simulink model "pfc_analog_test"  (R2021b)
settings: Solver=ode45  StartTime=0.0  StopTime=p.duration  MaxStep=p.max_step  RelTol=1e-8  AbsTol=1e-10
values from neighbouring files (symbols this model uses):
  config = [10 1514 1000]    [validate_m1.m]
  event_file = fullfile(folder,[name '_events.csv'])    [event_case.m]    (also in pfc_case.m)
  p = pfc_parameters();p.duration=0.08;p.load_step_time=1    [probe_closed_loop.m]    (also in validate_analog.m = pfc_parameters();p.duration=40e-6;p.max_step=2e-6; validate_control_reset.m = pfc_parameters())
settings Model: Creator=yangs  LastModifiedBy=yangs
settings SolverCC: ZeroCrossControl=EnableAll  ZeroCrossAlgorithm=Adaptive

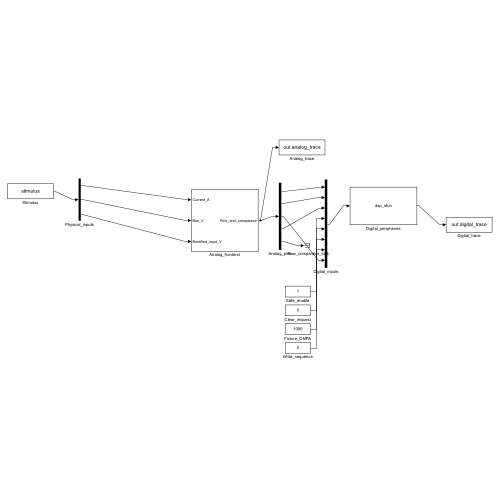
[thumbnail: Simulink's stored preview of the top-level diagram]
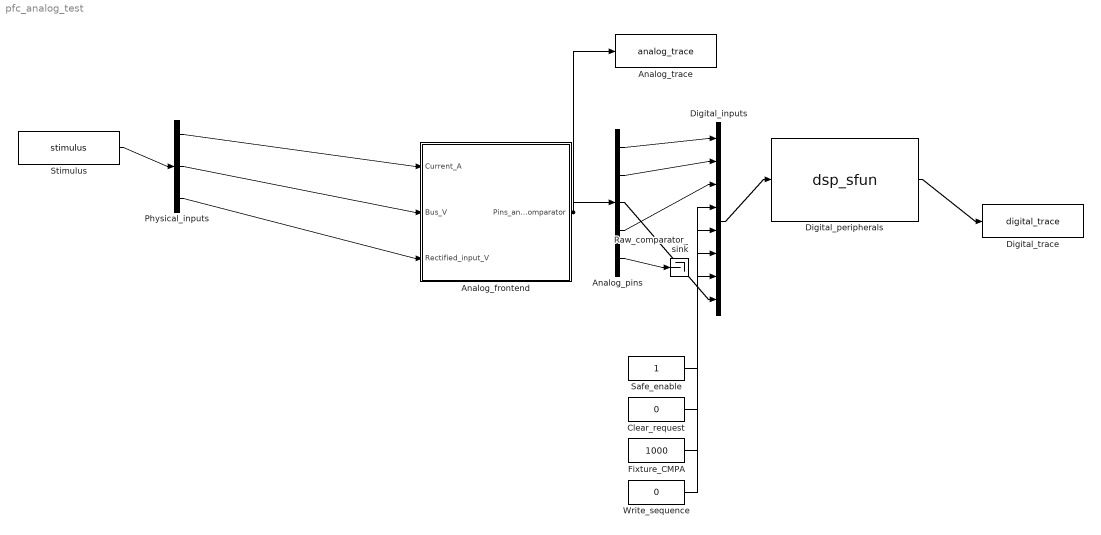
== system pfc_analog_test ==
  Analog_frontend : Subsystem
  Analog_pins : Demux  Outputs=5
  Analog_trace : ToWorkspace  VariableName=analog_trace  SaveFormat=Structure With Time  SampleTime=-1
  Clear_request : Constant  Value=0
  Digital_inputs : Mux  Inputs=8
  Digital_peripherals : S-Function  FunctionName=dsp_sfun  Parameters=config,event_file  SFunctionDeploymentMode=off  EnableBusSupport=off
  Digital_trace : ToWorkspace  VariableName=digital_trace  SaveFormat=Structure With Time  SampleTime=-1
  Fixture_CMPA : Constant  Value=1000
  Physical_inputs : Demux  Outputs=3
  Raw_comparator_sink : Terminator
  Safe_enable : Constant
  Stimulus : FromWorkspace  VariableName=stimulus  Interpolate=off  OutputAfterFinalValue=Holding final value
  Write_sequence : Constant  Value=0
  wires:
  Stimulus/1 -> Physical_inputs/1
  Analog_frontend/1(Pins_and_comparator) -> Analog_pins/1, Analog_trace/1
  Analog_pins/1 -> Digital_inputs/1
  Analog_pins/2 -> Digital_inputs/2
  Analog_pins/4 -> Digital_inputs/3
  Analog_pins/3 -> Digital_inputs/8
  Safe_enable/1 -> Digital_inputs/4
  Clear_request/1 -> Digital_inputs/5
  Fixture_CMPA/1 -> Digital_inputs/6
  Write_sequence/1 -> Digital_inputs/7
  Analog_pins/5 -> Raw_comparator_sink/1
  Digital_inputs/1 -> Digital_peripherals/1
  Digital_peripherals/1 -> Digital_trace/1
  Physical_inputs/1 -> Analog_frontend/1(Current_A)
  Physical_inputs/2 -> Analog_frontend/2(Bus_V)
  Physical_inputs/3 -> Analog_frontend/3(Rectified_input_V)

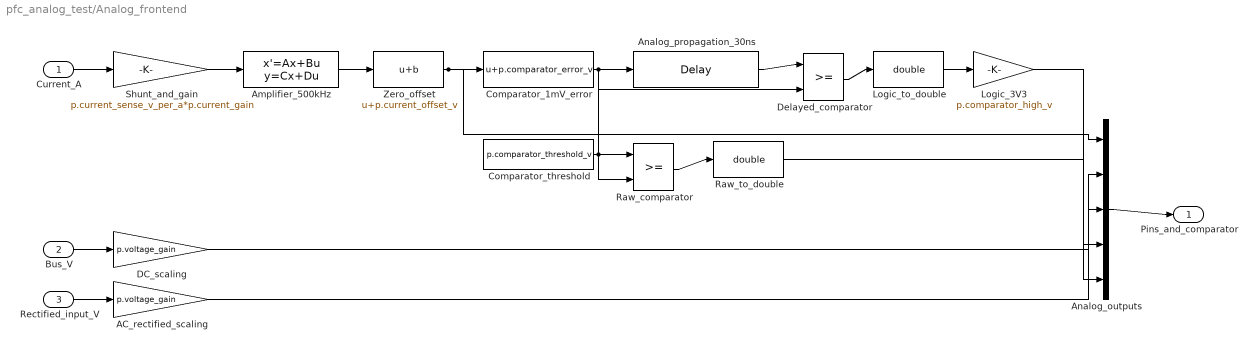
== system pfc_analog_test/Analog_frontend ==
  Current_A : Inport
  Bus_V : Inport  Port=2
  Rectified_input_V : Inport  Port=3
  AC_rectified_scaling : Gain  Gain=p.voltage_gain
  Amplifier_500kHz : StateSpace  A=-1/p.current_tau  B=1/p.current_tau  D=0  InitialCondition=0
  Analog_outputs : Mux  Inputs=5
  Analog_propagation_30ns : TransportDelay  DelayTime=p.comparator_delay_s
  Comparator_1mV_error : Bias  Bias=p.comparator_error_v
  Comparator_threshold : Constant  Value=p.comparator_threshold_v
  DC_scaling : Gain  Gain=p.voltage_gain
  Delayed_comparator : RelationalOperator  OutDataTypeStr=boolean  RndMeth=Simplest
  Logic_3V3 : Gain  Gain=p.comparator_high_v
  Logic_to_double : DataTypeConversion  OutDataTypeStr=double
  Raw_comparator : RelationalOperator  OutDataTypeStr=boolean  RndMeth=Simplest
  Raw_to_double : DataTypeConversion  OutDataTypeStr=double
  Shunt_and_gain : Gain  Gain=p.current_sense_v_per_a*p.current_gain
  Zero_offset : Bias  Bias=p.current_offset_v
  Pins_and_comparator : Outport
  wires:
  Current_A/1 -> Shunt_and_gain/1
  Shunt_and_gain/1 -> Amplifier_500kHz/1
  Amplifier_500kHz/1 -> Zero_offset/1
  Bus_V/1 -> DC_scaling/1
  Rectified_input_V/1 -> AC_rectified_scaling/1
  Zero_offset/1 -> Comparator_1mV_error/1, Analog_outputs/1
  Comparator_1mV_error/1 -> Analog_propagation_30ns/1, Raw_comparator/1
  Analog_propagation_30ns/1 -> Delayed_comparator/1
  Comparator_threshold/1 -> Delayed_comparator/2, Raw_comparator/2
  Delayed_comparator/1 -> Logic_to_double/1
  Logic_to_double/1 -> Logic_3V3/1
  Raw_comparator/1 -> Raw_to_double/1
  DC_scaling/1 -> Analog_outputs/2
  AC_rectified_scaling/1 -> Analog_outputs/3
  Logic_3V3/1 -> Analog_outputs/4
  Raw_to_double/1 -> Analog_outputs/5
  Analog_outputs/1 -> Pins_and_comparator/1
